simulink model "sensorFusion"  (R2025b)
settings: Solver=FixedStepAuto  StartTime=0.0  StopTime=10.0  RelTol=1e-3
settings Model: Creator=jakek  LastModifiedBy=jakek
settings SolverCC: AutoInsertRateTranBlk=on
settings OptimizationCC: EnhancedBackFolding=on  PassReuseOutputArgsAs=Individual arguments  ZeroExternalMemoryAtStartup=off  ZeroInternalMemoryAtStartup=off  MaxStackSize=64  OptimizeBlockOrder=speed  DifferentSizesBufferReuse=on  OptimizationCustomize=off  EfficientTunableParamExpr=on
settings DebuggingCC: ParameterTunabilityLossMsg=error
settings HardwareCC: ProdBitPerPointer=32.0  ProdBitPerSizeT=32.0  ProdBitPerPtrDiffT=32.0  ProdLargestAtomicInteger=Long  ProdLargestAtomicFloat=Double  ProdWordSize=32.0  ProdHWDeviceType=ARM Compatible->ARM Cortex
settings SFSimCC: MATLABDynamicMemAlloc=off  SimTargetLang=C++  SimDLTargetLibrary=mkl-dnn
settings RTWCC: SystemTargetFile=ert.tlc  GenCodeOnly=on  PackageGeneratedCodeAndArtifacts=on  TemplateMakefile=ert_default_tmf  GenerateReport=on  Toolchain=Arduino ARM M7  BuildConfiguration=Faster Runs  LaunchReport=on  TargetLang=C++  Description=Embedded Coder
settings CodeAppCC: ForceParamTrailComments=on  IgnoreCustomStorageClasses=off  OperatorAnnotations=on  SimulinkDataObjDesc=on  SFDataObjDesc=on  InsertBlockDesc=on
settings ERTTargetCC: ExtModeTransport=3.0  ExtModeStaticAlloc=on  ExtModeStaticAllocSize=65536.0  ExtModeMexFile=ext_xcp  ExtModeIntrfLevel=Level2 - Open  InlinedParameterPlacement=Hierarchical  RootIOFormat=Structure reference  ERTCustomFileTemplate=example_file_process.tlc  IndentStyle=Allman  IndentSize=4  TargetLangStandard=C++11 (ISO)  CodeInterfacePackaging=C++ class  SubcomponentCodeInterfacePackaging=C++ class  SupportContinuousTime=on  SupportVariableSizeSignals=on

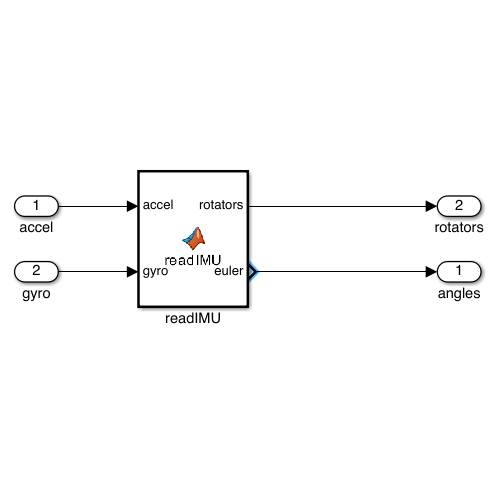
[thumbnail: Simulink's stored preview of the top-level diagram]
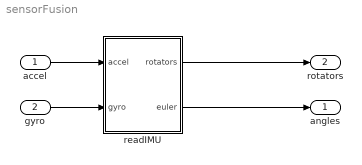
== system sensorFusion ==
  accel : Inport  PortDimensions=[1 3]
  gyro : Inport  Port=2  PortDimensions=[1 3]
  readIMU : MATLAB Function  TreatAsAtomicUnit=on
  angles : Outport  PortDimensions=[1 3]
  rotators : Outport  Port=2  PortDimensions=[1 4]
  wires:
  gyro/1 -> readIMU/2(gyro)
  accel/1 -> readIMU/1(accel)
  readIMU/1(rotators) -> rotators/1
  readIMU/2(euler) -> angles/1

== matlab function sensorFusion/readIMU ==
  data: rotators output; accel input; gyro input; euler output
function [rotators, euler] = readIMU(accel, gyro)
    arguments
        accel (1,3) double
        gyro (1,3) double
    end

    SampleRate = 50.0;

    persistent FUSE;    
    if isempty(FUSE)
        FUSE = imufilter("SampleRate", SampleRate);
    end

    quaternions = FUSE(accel, gyro);
    rotators = compact(quaternions);
    euler = quat2eul(quaternions);
    
end
